simulink model "anti_windup_simulink"  (R2022a)
settings: Solver=VariableStepAuto  StartTime=0.0  StopTime=2500  RelTol=1e-3
undefined symbols (not defined in the file): K_sys, Kp, sigbuilder_block, tau_sys, Td, theta_sys, Ti
settings Model: Creator=raha  LastModifiedBy=raha

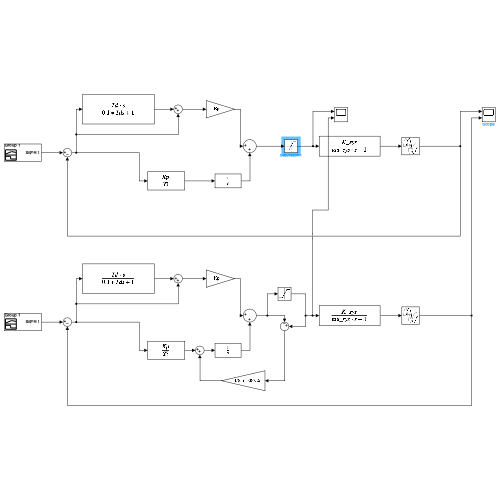
[thumbnail: Simulink's stored preview of the top-level diagram]
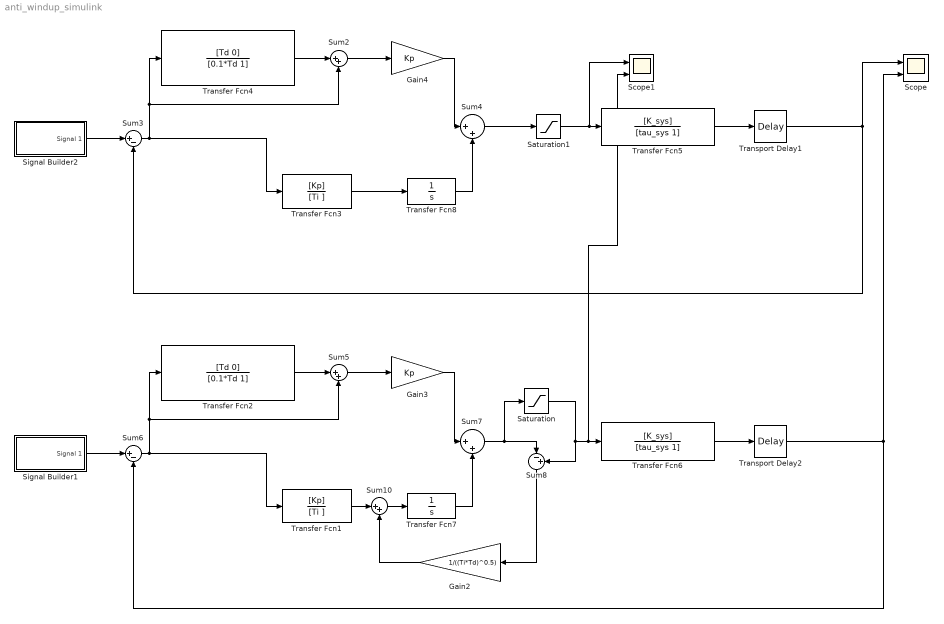
== system anti_windup_simulink ==
  Gain2 : Gain  Gain=1/((Ti*Td)^0.5)
  Gain3 : Gain  Gain=Kp
  Gain4 : Gain  Gain=Kp
  Saturation : Saturate  UpperLimit=100  LowerLimit=0
  Saturation1 : Saturate  UpperLimit=100  LowerLimit=0
  Scope : Scope  NumInputPorts=2
  Scope1 : Scope  NumInputPorts=2
  Signal Builder1 : Subsystem  Tag=STV Subsys  LoadFcn=sigbuilder_block('load');  StartFcn=sigbuilder_block('start');  StopFcn=sigbuilder_block('stop');  ClipboardFcn=sigbuilder_block('clipboard');  mask(Sigbuilder block){tuvar=[0:10]}
      mask help: Simulink:masks:SigbuilderBlock_MD
      mask init:
      | if ~strcmp(get_param(bdroot(gcbh),'SimulationStatus'),'stopped') tuvar = sigbuilder_block('maskInit'); end
      settings: CopyFcn=sigbuilder_block('copy');  DeleteFcn=sigbuilder_block('delete');  ModelCloseFcn=sigbuilder_block('modelClose');  PreSaveFcn=sigbuilder_block('preSave');  PauseFcn=sigbuilder_block('pause');  ContinueFcn=sigbuilder_block('continue');  NameChangeFcn=sigbuilder_block('namechange');  OpenFcn=sigbuilder_block('open',[437.6 199.2 550.4 400 ]);  CloseFcn=sigbuilder_block('close');
      mask Display: plot(0, 0, 100, 100,[2, 2, 32, 32, 2], [68, 8, 8, 68, 68],[32, 2], [38, 38], [32, 19, 2],[53, 60, 44], [32, 17, 17, 2],[16, 16, 31, 31]);txt = getActiveGroup(gcbh);text(2, 100, txt,'verticalAlignment', 'top');
  Signal Builder2 : Subsystem  Tag=STV Subsys  LoadFcn=sigbuilder_block('load');  StartFcn=sigbuilder_block('start');  StopFcn=sigbuilder_block('stop');  ClipboardFcn=sigbuilder_block('clipboard');  mask(Sigbuilder block){tuvar=[0:10]}
      mask help: Simulink:masks:SigbuilderBlock_MD
      mask init:
      | if ~strcmp(get_param(bdroot(gcbh),'SimulationStatus'),'stopped') tuvar = sigbuilder_block('maskInit'); end
      settings: CopyFcn=sigbuilder_block('copy');  DeleteFcn=sigbuilder_block('delete');  ModelCloseFcn=sigbuilder_block('modelClose');  PreSaveFcn=sigbuilder_block('preSave');  PauseFcn=sigbuilder_block('pause');  ContinueFcn=sigbuilder_block('continue');  NameChangeFcn=sigbuilder_block('namechange');  OpenFcn=sigbuilder_block('open',[437.6 199.2 550.4 400 ]);  CloseFcn=sigbuilder_block('close');
      mask Display: plot(0, 0, 100, 100,[2, 2, 32, 32, 2], [68, 8, 8, 68, 68],[32, 2], [38, 38], [32, 19, 2],[53, 60, 44], [32, 17, 17, 2],[16, 16, 31, 31]);txt = getActiveGroup(gcbh);text(2, 100, txt,'verticalAlignment', 'top');
  Sum{2,4..5,7,10} (5 alike) : Sum  Inputs=|++
  Sum3 : Sum  Inputs=|+-
  Sum6 : Sum  Inputs=|+-
  Sum8 : Sum  Inputs=|-+
  Transfer Fcn1 : TransferFcn  Numerator=[Kp]  Denominator=[Ti ]
  Transfer Fcn2 : TransferFcn  Numerator=[Td 0]  Denominator=[0.1*Td 1]
  Transfer Fcn3 : TransferFcn  Numerator=[Kp]  Denominator=[Ti ]
  Transfer Fcn4 : TransferFcn  Numerator=[Td 0]  Denominator=[0.1*Td 1]
  Transfer Fcn5 : TransferFcn  Numerator=[K_sys]  Denominator=[tau_sys 1]
  Transfer Fcn6 : TransferFcn  Numerator=[K_sys]  Denominator=[tau_sys 1]
  Transfer Fcn7 : TransferFcn  Denominator=[1 0]
  Transfer Fcn8 : TransferFcn  Denominator=[1 0]
  Transport Delay1 : TransportDelay  DelayTime=theta_sys
  Transport Delay2 : TransportDelay  DelayTime=theta_sys
  wires:
  Transfer Fcn2/1 -> Sum5/1
  Signal Builder1/1(Signal 1) -> Sum6/1
  Transport Delay2/1 -> Scope/2, Sum6/2
  Gain3/1 -> Sum7/1
  Transfer Fcn6/1 -> Transport Delay2/1
  Sum7/1 -> Sum8/1, Saturation/1
  Sum5/1 -> Gain3/1
  Saturation/1 -> Sum8/2, Scope1/2, Transfer Fcn6/1
  Sum10/1 -> Transfer Fcn7/1
  Transfer Fcn1/1 -> Sum10/1
  Sum8/1 -> Gain2/1
  Transfer Fcn7/1 -> Sum7/2
  Gain2/1 -> Sum10/2
  Sum6/1 -> Transfer Fcn2/1, Sum5/2, Transfer Fcn1/1
  Sum3/1 -> Transfer Fcn4/1, Sum2/2, Transfer Fcn3/1
  Signal Builder2/1(Signal 1) -> Sum3/1
  Transfer Fcn4/1 -> Sum2/1
  Transfer Fcn3/1 -> Transfer Fcn8/1
  Sum4/1 -> Saturation1/1
  Transfer Fcn8/1 -> Sum4/2
  Sum2/1 -> Gain4/1
  Transfer Fcn5/1 -> Transport Delay1/1
  Gain4/1 -> Sum4/1
  Transport Delay1/1 -> Scope/1, Sum3/2
  Saturation1/1 -> Scope1/1, Transfer Fcn5/1

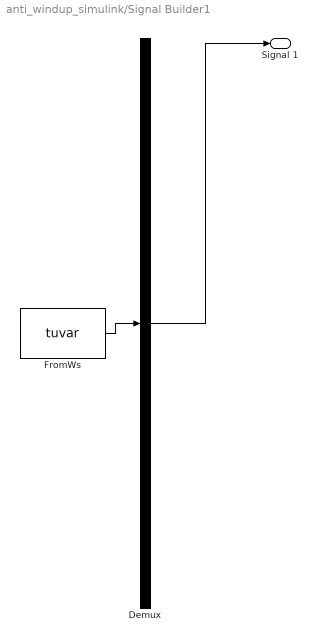
== system anti_windup_simulink/Signal Builder1 ==
  Demux : Demux  Tag=STV Demux  Outputs=1
      settings: DisplayOption=none
  FromWs : FromWorkspace  Tag=STV FromWs  VariableName=tuvar
      SigBuilderData=|
      | common.afterFinalStr = 'Extrapolate'
      | common.sampleTime = 0
      | dataSet.timeRange = [0 3500]
      | dataSet.name = 'Group 1'
      | sbobj.Groups.Name = 'Group 1'
      | sbobj.Groups.Signals.Name = 'Signal 1'
      | sbobj.Groups.Signals.XData = [0 620 620 1700 1700 3500]
      | sbobj.Groups.Signals.YData = [35 35 135 135 35 35]
      | sbobj.Groups.TimeRange = [0 3500]
  Signal 1 : Outport  Tag=STV Outport
  wires:
  Demux/1 -> Signal 1/1
  FromWs/1 -> Demux/1

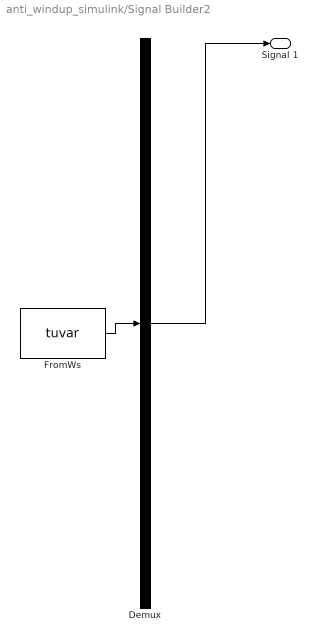
== system anti_windup_simulink/Signal Builder2 ==
  Demux : Demux  Tag=STV Demux  Outputs=1
      settings: DisplayOption=none
  FromWs : FromWorkspace  Tag=STV FromWs  VariableName=tuvar
      SigBuilderData=|
      | common.afterFinalStr = 'Extrapolate'
      | common.sampleTime = 0
      | dataSet.timeRange = [0 3500]
      | dataSet.name = 'Group 1'
      | sbobj.Groups.Name = 'Group 1'
      | sbobj.Groups.Signals.Name = 'Signal 1'
      | sbobj.Groups.Signals.XData = [0 620 620 1700 1700 3500]
      | sbobj.Groups.Signals.YData = [35 35 135 135 35 35]
      | sbobj.Groups.TimeRange = [0 3500]
  Signal 1 : Outport  Tag=STV Outport
  wires:
  Demux/1 -> Signal 1/1
  FromWs/1 -> Demux/1
